simulink model "uacs_manual_pid"  (R2024a)
settings: Solver=ode4  StartTime=0.0  StopTime=sim_t_end  FixedStep=sim_ts_ctrl  RelTol=1e-3
undefined symbols (not defined in the file): DiscIntNeverNeededParam, sim_c_neg1, sim_c_zero, sim_flight_mode, sim_G_surf, sim_pid_h_Dden, sim_pid_h_Dnum_abs, sim_pid_h_Isat, sim_pid_h_Isat_neg, sim_pid_h_Kp_abs, sim_pid_h_lim, sim_pid_h_lim_neg, sim_pid_h_pol, sim_pid_h_Ts, sim_pid_p_Dden, sim_pid_p_Dnum_abs, sim_pid_p_Isat, sim_pid_p_Isat_neg, sim_pid_p_Kp_abs, sim_pid_p_pol, sim_pid_p_Ts, sim_pid_phi_Dden, sim_pid_phi_Dnum_abs, sim_pid_phi_Isat, sim_pid_phi_Isat_neg, sim_pid_phi_Kp_abs, sim_pid_phi_pol, sim_pid_phi_Ts, sim_pid_q_Dden, sim_pid_q_Dnum_abs, sim_pid_q_Isat, sim_pid_q_Isat_neg, sim_pid_q_Kp_abs, sim_pid_q_pol, sim_pid_q_Ts, sim_pid_r_Dden, sim_pid_r_Dnum_abs, sim_pid_r_Isat, sim_pid_r_Isat_neg, sim_pid_r_Kp_abs, sim_pid_r_pol, sim_pid_r_Ts, sim_pid_theta_Dden, sim_pid_theta_Dnum_abs, sim_pid_theta_Isat, sim_pid_theta_Isat_neg, sim_pid_theta_Kp_abs, sim_pid_theta_pol, sim_pid_theta_Ts, sim_pid_V_Dden, sim_pid_V_Dnum_abs, sim_pid_V_Isat, sim_pid_V_Isat_neg, sim_pid_V_Kp_abs, sim_pid_V_pol, sim_pid_V_Ts, sim_rate_cmd_lim_p, sim_rate_cmd_lim_q, sim_rate_cmd_lim_r, sim_T_trim ... (+1)
settings Model: Creator=Ash Trailer  LastModifiedBy=Ash Trailer
settings DataIOCC: SaveFormat=StructureWithTime
settings DebuggingCC: AlgebraicLoopMsg=error

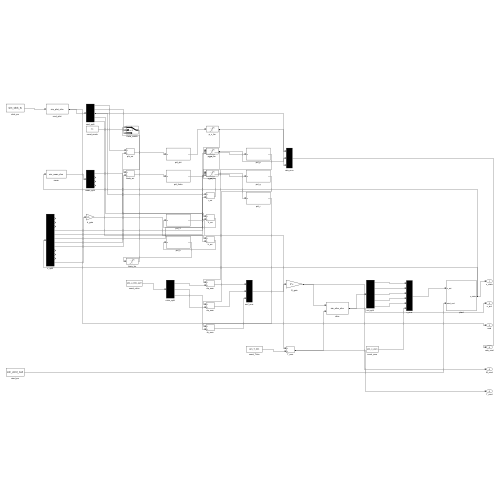
[thumbnail: Simulink's stored preview of the top-level diagram]
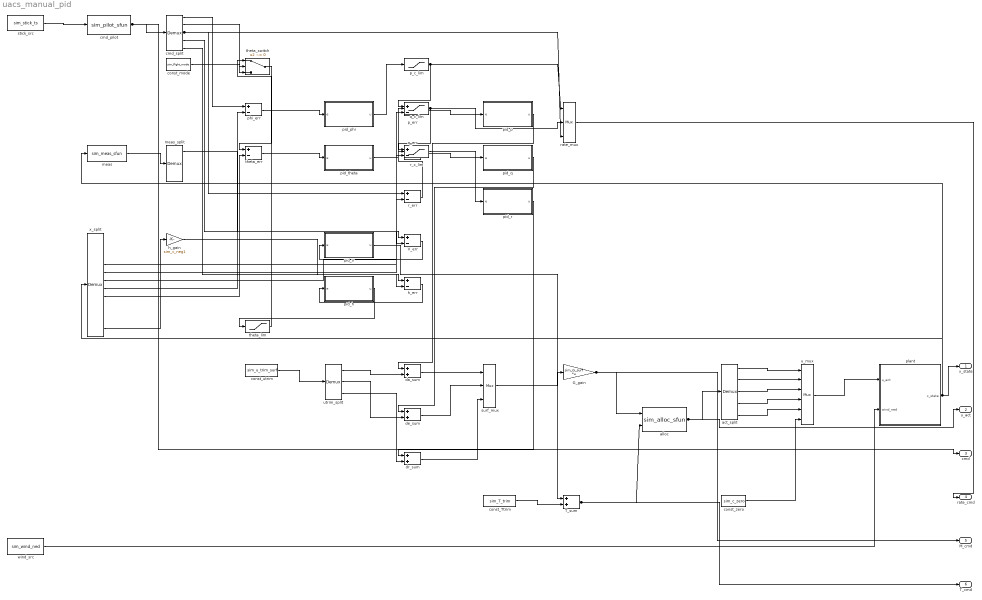
== system uacs_manual_pid ==
  G_gain : Gain  Gain=sim_G_surf  Multiplication=Matrix(K*u)
  T_sum : Sum
  V_err : Sum  Inputs=+-
  act_split : Demux  Outputs=5
  alloc : M-S-Function  FunctionName=sim_alloc_sfun
  cmd_pilot : M-S-Function  FunctionName=sim_pilot_sfun
  cmd_split : Demux  Outputs=5
  const_Ttrim : Constant  Value=sim_T_trim
  const_mode : Constant  Value=sim_flight_mode
  const_utrim : Constant  Value=sim_u_trim_surf
  const_zero : Constant  Value=sim_c_zero
  da_sum : Sum
  de_sum : Sum
  dr_sum : Sum
  h_err : Sum  Inputs=+-
  h_gain : Gain  Gain=sim_c_neg1
  meas : M-S-Function  FunctionName=sim_meas_sfun
  meas_split : Demux
  p_c_lim : Saturate  UpperLimit=sim_rate_cmd_lim_p  LowerLimit=-sim_rate_cmd_lim_p
  p_err : Sum  Inputs=+-
  phi_err : Sum  Inputs=+-
  pid_V : Subsystem
  pid_h : Subsystem
  pid_p : Subsystem
  pid_phi : Subsystem
  pid_q : Subsystem
  pid_r : Subsystem
  pid_theta : Subsystem
  plant : Subsystem
  q_c_lim : Saturate  UpperLimit=sim_rate_cmd_lim_q  LowerLimit=-sim_rate_cmd_lim_q
  q_err : Sum  Inputs=+-
  r_c_lim : Saturate  UpperLimit=sim_rate_cmd_lim_r  LowerLimit=-sim_rate_cmd_lim_r
  r_err : Sum  Inputs=+-
  rate_mux : Mux  Inputs=3
  stick_src : FromWorkspace  VariableName=sim_stick_ts  OutputAfterFinalValue=Holding final value
  surf_mux : Mux  Inputs=3
  theta_err : Sum  Inputs=+-
  theta_lim : Saturate  UpperLimit=sim_pid_h_lim  LowerLimit=sim_pid_h_lim_neg
  theta_switch : Switch  Criteria=u2 ~= 0  Threshold=sim_c_zero  SaturateOnIntegerOverflow=off  InputSameDT=off
  u_mux : Mux  Inputs=6
  utrim_split : Demux  Outputs=3
  wind_src : FromWorkspace  VariableName=sim_wind_ned  OutputAfterFinalValue=Holding final value
  x_split : Demux  Outputs=12
  x_state : Outport
  u_act : Outport  Port=2
  cmd : Outport  Port=3
  rate_cmd : Outport  Port=4
  M_cmd : Outport  Port=5
  T_cmd : Outport  Port=6
  wires:
  stick_src/1 -> cmd_pilot/1
  cmd_pilot/1 -> cmd_split/1, cmd/1
  cmd_split/1 -> phi_err/1
  cmd_split/2 -> theta_switch/3
  cmd_split/3 -> r_err/1, rate_mux/3
  cmd_split/4 -> V_err/1
  cmd_split/5 -> h_err/1
  const_mode/1 -> theta_switch/2
  theta_lim/1 -> theta_switch/1
  theta_switch/1 -> theta_err/1
  phi_err/1 -> pid_phi/1(e)
  pid_phi/1(u) -> p_c_lim/1
  p_c_lim/1 -> p_err/1, rate_mux/1
  p_err/1 -> pid_p/1(e)
  pid_p/1(u) -> da_sum/1
  theta_err/1 -> pid_theta/1(e)
  pid_theta/1(u) -> q_c_lim/1
  q_c_lim/1 -> q_err/1, rate_mux/2
  q_err/1 -> pid_q/1(e)
  pid_q/1(u) -> de_sum/1
  r_err/1 -> r_c_lim/1
  r_c_lim/1 -> pid_r/1(e)
  pid_r/1(u) -> dr_sum/1
  V_err/1 -> pid_V/1(e)
  pid_V/1(u) -> T_sum/1
  h_err/1 -> pid_h/1(e)
  pid_h/1(u) -> theta_lim/1
  rate_mux/1 -> rate_cmd/1
  const_utrim/1 -> utrim_split/1
  utrim_split/1 -> da_sum/2
  utrim_split/2 -> de_sum/2
  utrim_split/3 -> dr_sum/2
  da_sum/1 -> surf_mux/1
  de_sum/1 -> surf_mux/2
  dr_sum/1 -> surf_mux/3
  surf_mux/1 -> G_gain/1
  G_gain/1 -> alloc/1, M_cmd/1
  const_Ttrim/1 -> T_sum/2
  T_sum/1 -> alloc/2, T_cmd/1
  alloc/1 -> act_split/1, u_act/1
  act_split/1 -> u_mux/1
  act_split/2 -> u_mux/2
  act_split/3 -> u_mux/3
  act_split/4 -> u_mux/4
  act_split/5 -> u_mux/5
  const_zero/1 -> u_mux/6
  u_mux/1 -> plant/1(u_act)
  wind_src/1 -> plant/2(wind_ned)
  plant/1(x_state) -> x_state/1, x_split/1, meas/1
  meas/1 -> meas_split/1
  meas_split/1 -> V_err/2
  x_split/4 -> p_err/2
  x_split/5 -> q_err/2
  x_split/6 -> r_err/2
  x_split/7 -> phi_err/2
  x_split/8 -> theta_err/2
  x_split/12 -> h_gain/1
  h_gain/1 -> h_err/2

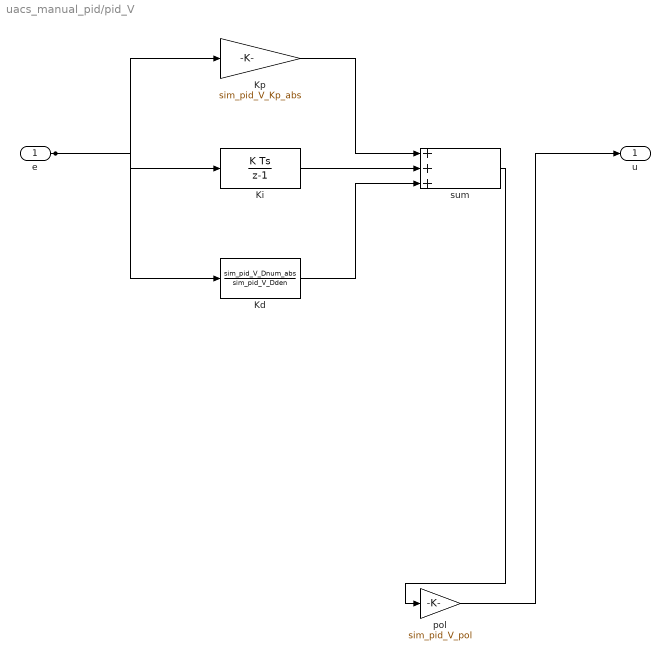
== system uacs_manual_pid/pid_V ==
  e : Inport
  Kd : DiscreteTransferFcn  Numerator=sim_pid_V_Dnum_abs  Denominator=sim_pid_V_Dden  SampleTime=sim_pid_V_Ts
  Ki : DiscreteIntegrator  gainval=sim_pid_V_Ki_abs  SampleTime=sim_pid_V_Ts  LimitOutput=on  UpperSaturationLimit=sim_pid_V_Isat  LowerSaturationLimit=sim_pid_V_Isat_neg  ICPrevOutput=DiscIntNeverNeededParam  ICPrevScaledInput=DiscIntNeverNeededParam
  Kp : Gain  Gain=sim_pid_V_Kp_abs
  pol : Gain  Gain=sim_pid_V_pol
  sum : Sum  Inputs=+++
  u : Outport
  wires:
  e/1 -> Kp/1, Ki/1, Kd/1
  Kp/1 -> sum/1
  Ki/1 -> sum/2
  Kd/1 -> sum/3
  sum/1 -> pol/1
  pol/1 -> u/1

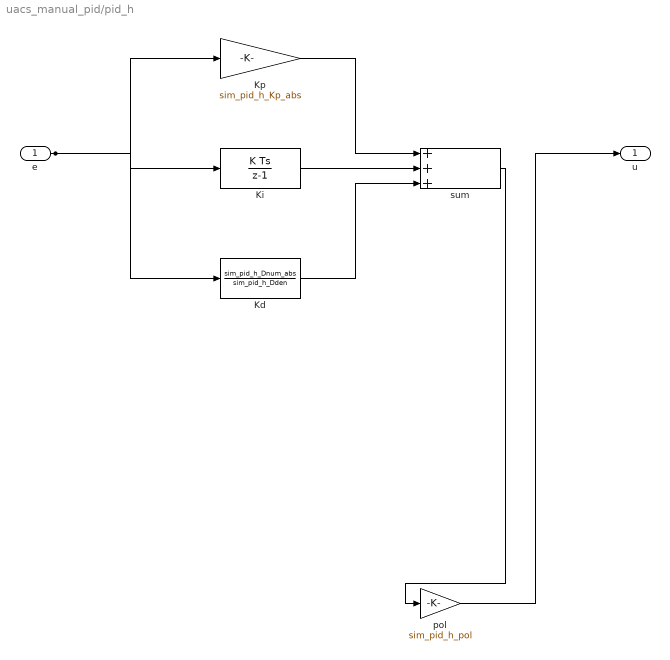
== system uacs_manual_pid/pid_h ==
  e : Inport
  Kd : DiscreteTransferFcn  Numerator=sim_pid_h_Dnum_abs  Denominator=sim_pid_h_Dden  SampleTime=sim_pid_h_Ts
  Ki : DiscreteIntegrator  gainval=sim_pid_h_Ki_abs  SampleTime=sim_pid_h_Ts  LimitOutput=on  UpperSaturationLimit=sim_pid_h_Isat  LowerSaturationLimit=sim_pid_h_Isat_neg  ICPrevOutput=DiscIntNeverNeededParam  ICPrevScaledInput=DiscIntNeverNeededParam
  Kp : Gain  Gain=sim_pid_h_Kp_abs
  pol : Gain  Gain=sim_pid_h_pol
  sum : Sum  Inputs=+++
  u : Outport
  wires:
  e/1 -> Kp/1, Ki/1, Kd/1
  Kp/1 -> sum/1
  Ki/1 -> sum/2
  Kd/1 -> sum/3
  sum/1 -> pol/1
  pol/1 -> u/1

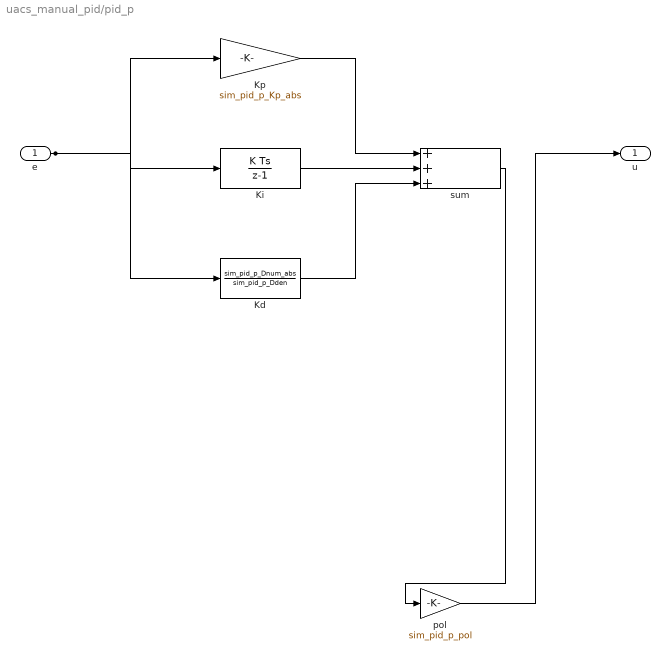
== system uacs_manual_pid/pid_p ==
  e : Inport
  Kd : DiscreteTransferFcn  Numerator=sim_pid_p_Dnum_abs  Denominator=sim_pid_p_Dden  SampleTime=sim_pid_p_Ts
  Ki : DiscreteIntegrator  gainval=sim_pid_p_Ki_abs  SampleTime=sim_pid_p_Ts  LimitOutput=on  UpperSaturationLimit=sim_pid_p_Isat  LowerSaturationLimit=sim_pid_p_Isat_neg  ICPrevOutput=DiscIntNeverNeededParam  ICPrevScaledInput=DiscIntNeverNeededParam
  Kp : Gain  Gain=sim_pid_p_Kp_abs
  pol : Gain  Gain=sim_pid_p_pol
  sum : Sum  Inputs=+++
  u : Outport
  wires:
  e/1 -> Kp/1, Ki/1, Kd/1
  Kp/1 -> sum/1
  Ki/1 -> sum/2
  Kd/1 -> sum/3
  sum/1 -> pol/1
  pol/1 -> u/1

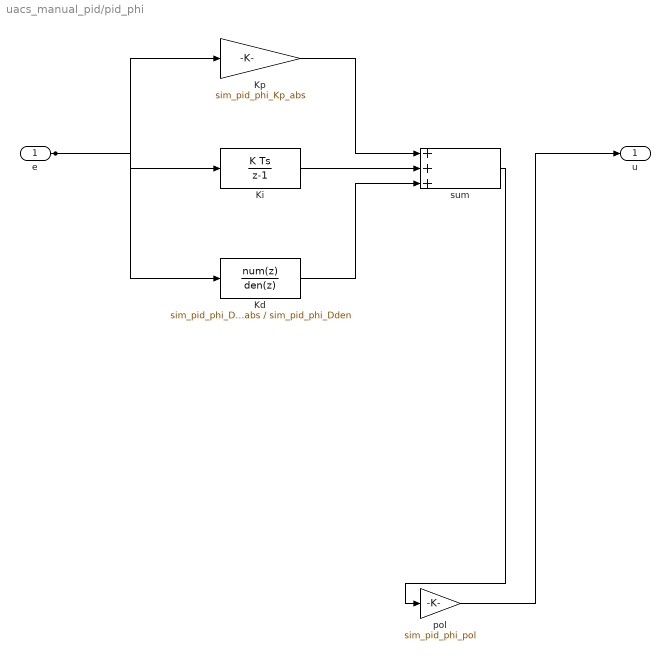
== system uacs_manual_pid/pid_phi ==
  e : Inport
  Kd : DiscreteTransferFcn  Numerator=sim_pid_phi_Dnum_abs  Denominator=sim_pid_phi_Dden  SampleTime=sim_pid_phi_Ts
  Ki : DiscreteIntegrator  gainval=sim_pid_phi_Ki_abs  SampleTime=sim_pid_phi_Ts  LimitOutput=on  UpperSaturationLimit=sim_pid_phi_Isat  LowerSaturationLimit=sim_pid_phi_Isat_neg  ICPrevOutput=DiscIntNeverNeededParam  ICPrevScaledInput=DiscIntNeverNeededParam
  Kp : Gain  Gain=sim_pid_phi_Kp_abs
  pol : Gain  Gain=sim_pid_phi_pol
  sum : Sum  Inputs=+++
  u : Outport
  wires:
  e/1 -> Kp/1, Ki/1, Kd/1
  Kp/1 -> sum/1
  Ki/1 -> sum/2
  Kd/1 -> sum/3
  sum/1 -> pol/1
  pol/1 -> u/1

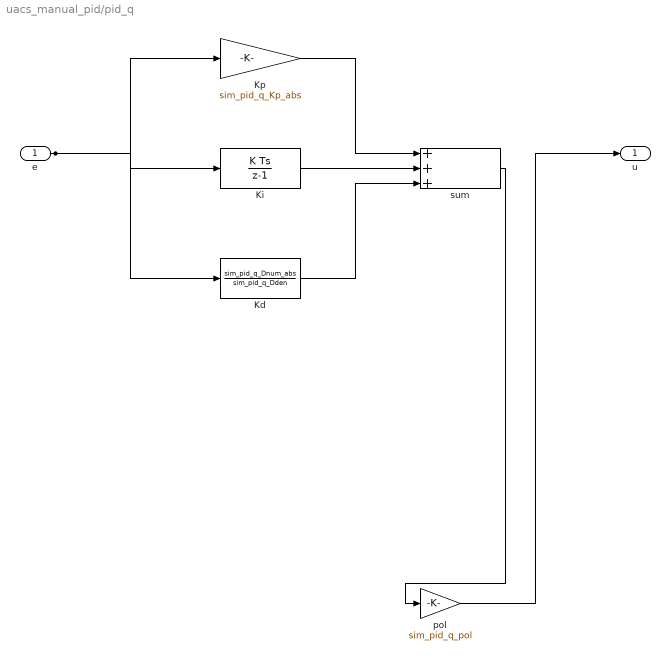
== system uacs_manual_pid/pid_q ==
  e : Inport
  Kd : DiscreteTransferFcn  Numerator=sim_pid_q_Dnum_abs  Denominator=sim_pid_q_Dden  SampleTime=sim_pid_q_Ts
  Ki : DiscreteIntegrator  gainval=sim_pid_q_Ki_abs  SampleTime=sim_pid_q_Ts  LimitOutput=on  UpperSaturationLimit=sim_pid_q_Isat  LowerSaturationLimit=sim_pid_q_Isat_neg  ICPrevOutput=DiscIntNeverNeededParam  ICPrevScaledInput=DiscIntNeverNeededParam
  Kp : Gain  Gain=sim_pid_q_Kp_abs
  pol : Gain  Gain=sim_pid_q_pol
  sum : Sum  Inputs=+++
  u : Outport
  wires:
  e/1 -> Kp/1, Ki/1, Kd/1
  Kp/1 -> sum/1
  Ki/1 -> sum/2
  Kd/1 -> sum/3
  sum/1 -> pol/1
  pol/1 -> u/1

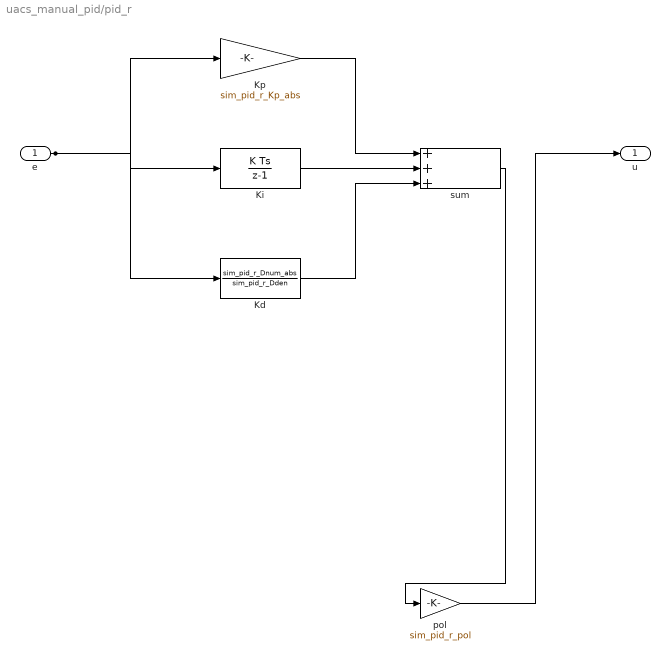
== system uacs_manual_pid/pid_r ==
  e : Inport
  Kd : DiscreteTransferFcn  Numerator=sim_pid_r_Dnum_abs  Denominator=sim_pid_r_Dden  SampleTime=sim_pid_r_Ts
  Ki : DiscreteIntegrator  gainval=sim_pid_r_Ki_abs  SampleTime=sim_pid_r_Ts  LimitOutput=on  UpperSaturationLimit=sim_pid_r_Isat  LowerSaturationLimit=sim_pid_r_Isat_neg  ICPrevOutput=DiscIntNeverNeededParam  ICPrevScaledInput=DiscIntNeverNeededParam
  Kp : Gain  Gain=sim_pid_r_Kp_abs
  pol : Gain  Gain=sim_pid_r_pol
  sum : Sum  Inputs=+++
  u : Outport
  wires:
  e/1 -> Kp/1, Ki/1, Kd/1
  Kp/1 -> sum/1
  Ki/1 -> sum/2
  Kd/1 -> sum/3
  sum/1 -> pol/1
  pol/1 -> u/1

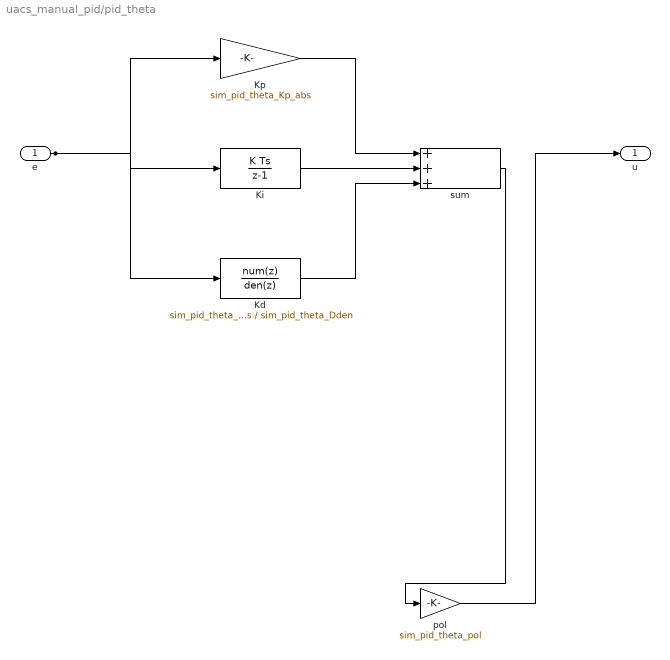
== system uacs_manual_pid/pid_theta ==
  e : Inport
  Kd : DiscreteTransferFcn  Numerator=sim_pid_theta_Dnum_abs  Denominator=sim_pid_theta_Dden  SampleTime=sim_pid_theta_Ts
  Ki : DiscreteIntegrator  gainval=sim_pid_theta_Ki_abs  SampleTime=sim_pid_theta_Ts  LimitOutput=on  UpperSaturationLimit=sim_pid_theta_Isat  LowerSaturationLimit=sim_pid_theta_Isat_neg  ICPrevOutput=DiscIntNeverNeededParam  ICPrevScaledInput=DiscIntNeverNeededParam
  Kp : Gain  Gain=sim_pid_theta_Kp_abs
  pol : Gain  Gain=sim_pid_theta_pol
  sum : Sum  Inputs=+++
  u : Outport
  wires:
  e/1 -> Kp/1, Ki/1, Kd/1
  Kp/1 -> sum/1
  Ki/1 -> sum/2
  Kd/1 -> sum/3
  sum/1 -> pol/1
  pol/1 -> u/1

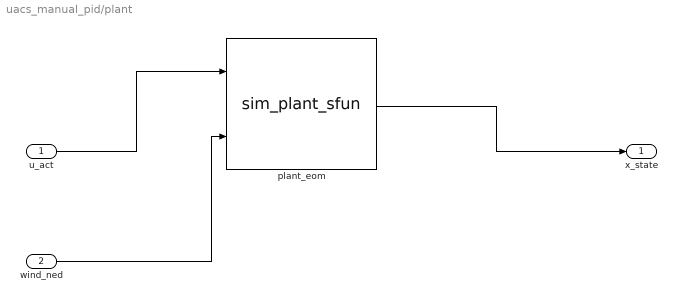
== system uacs_manual_pid/plant ==
  u_act : Inport
  wind_ned : Inport  Port=2
  plant_eom : M-S-Function  FunctionName=sim_plant_sfun
  x_state : Outport
  wires:
  u_act/1 -> plant_eom/1
  wind_ned/1 -> plant_eom/2
  plant_eom/1 -> x_state/1
